simulink model "RBSdev"  (R2024a)
settings: Solver=VariableStepAuto  StartTime=0.0  StopTime=10.0  RelTol=1e-3
undefined symbols (not defined in the file): I_charge_max, Id, Id_char, Imax, Ion, Iq, lambda, Ld, Lithium, Lq, p, Rs, Soc_max, Tmax, V_batt, Vdc_nom, Vs_max
libraries: mcbcontrolslib x4, spsBatteryLib x1, simulink x1, spsPermanentMagnetSynchronousMachineLib x1, spsSeriesRLCBranchLib x1, spsThreePhaseFaultLib x1, spsUniversalBridgeLib x1, spspowerguiLib x1
(part 2 of 2)

== matlab function RBSdev/Operation mode & reference determination/Mode Determination + (dq) references genration/High Speed (FW + MTPV logic)/mode 2 (MTPV +FW logic)/If Action Subsystem/MATLAB Function ==
  data: T_ref input; Id_ref output; Vs_max input; omega_e input; Rs input; Ld input; Lq input; lambda_pm input; I_max input; Iq_ref output
function [Id_ref, Iq_ref] = calculate_fw_currents(T_ref, Vs_max, omega_e, Rs, Ld, Lq, lambda_pm, I_max)
    % Field Weakening with current limit intersection
    
    delta_L = Ld - Lq;
    T_norm = T_ref / 1.5;
    
    % Iterate to find Id, Iq that satisfy both torque and voltage equations
    Id_guess = 0;
    Iq_guess = T_norm / lambda_pm;
    
    for iter = 1:100
        % Voltage equations
        Vd = Rs*Id_guess - omega_e*Lq*Iq_guess;
        Vq = Rs*Iq_guess + omega_e*Ld*Id_guess + omega_e*lambda_pm;
        Vs = sqrt(Vd^2 + Vq^2);
        
        % Torque
        T_calc = lambda_pm * Iq_guess + delta_L * Id_guess * Iq_guess;
        
        % Errors
        err_V = Vs - Vs_max;
        err_T = T_calc - T_norm;
        
        % Adjust Id (more negative = more FW)
        dId = -0.5;
        Vd_plus = Rs*(Id_guess+dId) - omega_e*Lq*Iq_guess;
        Vq_plus = Rs*Iq_guess + omega_e*Ld*(Id_guess+dId) + omega_e*lambda_pm;
        Vs_plus = sqrt(Vd_plus^2 + Vq_plus^2);
        dVs_dId = (Vs_plus - Vs) / dId;
        
        if abs(dVs_dId) > 1e-10
            Id_guess = Id_guess - err_V / dVs_dId;
        end
        
        % Adjust Iq to maintain torque
        if abs(delta_L * Id_guess) > 1e-10
            Iq_guess = T_norm / (lambda_pm + delta_L * Id_guess);
        else
            Iq_guess = T_norm / lambda_pm;
        end
        
        % Apply current limit
        Is = sqrt(Id_guess^2 + Iq_guess^2);
        if Is > I_max
            scale = I_max / Is;
            Id_guess = Id_guess * scale;
            Iq_guess = Iq_guess * scale;
        end
        
        if abs(err_V) < 0.1 && abs(err_T) < 0.01
            break;
        end
    end
    
    Id_ref = Id_guess;
    Iq_ref = Iq_guess;
end

== matlab function RBSdev/Field oriented control/PIcontrol & voltage calc ==
  data: Vd output; Id_ref input; Id input; Iq_ref input; Iq input; Vq output
function [Vd,Vq] = Current_PI_control_VoltageCalc(Id_ref,Id,Iq_ref,Iq)

    % ----- 6.5 FOC CURRENT CONTROL (PI Controllers) -----
    
    % Anti-windup limits
    Vd_max = Vs_max;
    Vq_max = Vs_max;
    
    % d-axis current error and PI
    err_Id = Id_ref - Id;
    int_err_Id = int_err_Id + err_Id * dt;
    
    % Anti-windup
    Vd_cmd = Kp_d * err_Id + Ki_d * int_err_Id;
    if abs(Vd_cmd) > Vd_max
        int_err_Id = int_err_Id - err_Id * dt;  % Revert integration
        Vd_cmd = sign(Vd_cmd) * Vd_max;
    end
    
    % q-axis current error and PI
    err_Iq = Iq_ref - Iq;
    int_err_Iq = int_err_Iq + err_Iq * dt;
    
    % Anti-windup
    Vq_cmd = Kp_q * err_Iq + Ki_q * int_err_Iq;
    if abs(Vq_cmd) > Vq_max
        int_err_Iq = int_err_Iq - err_Iq * dt;  % Revert integration
        Vq_cmd = sign(Vq_cmd) * Vq_max;
    end
    
    % Voltage limiting (circle constraint)
    Vs_cmd = sqrt(Vd_cmd^2 + Vq_cmd^2);
    if Vs_cmd > Vs_max
        Vd_cmd = Vd_cmd * Vs_max / Vs_cmd;
        Vq_cmd = Vq_cmd * Vs_max / Vs_cmd;
    end
    
    Vd = Vd_cmd;
    Vq = Vq_cmd;
    
end

== matlab function RBSdev/Field oriented control/SVPWM algo ==
  data: v_alpha input; d_a output; v_beta input; Vdc input; apply_saturation input; d_b output; d_c output
function [d_a, d_b, d_c] = svpwm_step(v_alpha, v_beta, Vdc, apply_saturation)
% SVPWM_STEP - Space Vector PWM duty cycle generation
%
% Inputs:
%   v_alpha          : Alpha-axis voltage reference [V]
%   v_beta           : Beta-axis voltage reference [V]
%   Vdc              : DC bus voltage [V]
%   apply_saturation : 1 = scale vector to linear region, 0 = skip
%
% Outputs:
%   d_a    : Phase A duty cycle [0 to 1]
%   d_b    : Phase B duty cycle [0 to 1]
%   d_c    : Phase C duty cycle [0 to 1]
%   overmod: Overmodulation flag (1 = exceeded linear region)
%   scale  : Scaling factor applied (1.0 = no scaling)

    %% Input protection
    if Vdc <= 0
        error('Vdc must be greater than 0');
    end

    %% Step 1 — Voltage Saturation (optional)
    v_lim = Vdc / sqrt(3);
    mag   = sqrt(v_alpha^2 + v_beta^2);

    if apply_saturation && mag > v_lim && mag > 1e-12
        scale       = v_lim / mag;
        v_alpha_use = v_alpha * scale;
        v_beta_use  = v_beta  * scale;
    else
        scale       = 1.0;
        v_alpha_use = v_alpha;
        v_beta_use  = v_beta;
    end

    %% Step 2 — Alpha-Beta to ABC (line-neutral references)
    v_a =  v_alpha_use;
    v_b = -0.5 * v_alpha_use + (sqrt(3)/2) * v_beta_use;
    v_c = -0.5 * v_alpha_use - (sqrt(3)/2) * v_beta_use;

    %% Step 3 — Zero-sequence injection (SVPWM offset)
    v_max = max([v_a, v_b, v_c]);
    v_min = min([v_a, v_b, v_c]);
    v_0   = -0.5 * (v_max + v_min);

    v_a0 = v_a + v_0;
    v_b0 = v_b + v_0;
    v_c0 = v_c + v_0;

    %% Step 4 — Duty cycle mapping
    d_a_raw = 0.5 + (v_a0 / Vdc);
    d_b_raw = 0.5 + (v_b0 / Vdc);
    d_c_raw = 0.5 + (v_c0 / Vdc);

    %% Step 6 — Clamp duties to [0, 1]
    d_a = min(max(d_a_raw, 0), 1);
    d_b = min(max(d_b_raw, 0), 1);
    d_c = min(max(d_c_raw, 0), 1);

end
